simulink model "PLL1"  (R2021b)
settings: Solver=ode45  StartTime=0.0  StopTime=500*synM/synFr  FixedStep=1/(3*synFr*synN/synM)  MaxStep=.5/(synFr*synN/synM)  RelTol=1e-3  EnableMultiTasking=on
PreLoadFcn:
  | synM = 3;    % frequency division ratio
  | synN = 10;   % frequency division ratio
  | synFr = 30e6;   % reference frequency
  | synFq = synFr;       % quiescent frequency
  | synSen = 40e6;   % VCO sensitivity
libraries: commblksprivate x3, dsparch4 x1, commsynccomp2 x1
Description:
  | Phase-Locked Loop (PLL)  Based Frequency Synthesis
  | 
  | This model shows how to simulate a phase-locked loop (PLL) frequency synthesizer.
settings Model: Creator=The MathWorks, Inc.  LastModifiedBy=think
settings SolverCC: AlgebraicLoopSolver=TrustRegion
settings DataIOCC: LimitDataPoints=on  SaveFormat=Array  SaveOutput=off  SaveTime=off  ReturnWorkspaceOutputs=off  SignalLoggingName=synSigsOut
settings OptimizationCC: BlockReduction=off  BooleanDataType=off  ExpressionDepthLimit=2147483647  InitFltsAndDblsToZero=on  EfficientMapNaN2IntZero=off  LifeSpan=inf
settings DebuggingCC: SaveWithParameterizedLinksMsg=none  UnderspecifiedInitializationDetection=Classic  MergeDetectMultiDrivingBlocksExec=none  CheckExecutionContextPreStartOutputMsg=on  SignalResolutionControl=TryResolveAllWithWarning  MultiTaskDSMMsg=warning  MultiTaskCondExecSysMsg=none  SigSpecEnsureSampleTimeMsg=none  FcnCallInpInsideContextMsg=warning  AllowSymbolicDim=off  StateNameClashWarn=warning  SFUnexpectedBacktrackingDiag=warning  SFNoUnconditionalDefaultTransitionDiag=warning  SFMachineParentedDataDiag=warning  ArithmeticOperatorsInVariantConditions=warning
settings HardwareCC: ProdBitPerPointer=32  ProdBitPerSizeT=32  ProdBitPerPtrDiffT=32  ProdLargestAtomicFloat=None  ProdIntDivRoundTo=Undefined  ProdEndianess=Unspecified  ProdWordSize=32  ProdHWDeviceType=32-bit Generic  TargetUnknown=on
settings ModelReferenceCC: UpdateModelReferenceTargets=IfOutOfDate  PropagateSignalLabelsOutOfModel=off
settings SFSimCC: SimUseLocalCustomCode=off  CustomCodeUndefinedFunction=UseInterfaceOnly
settings RTWCC: RTWUseLocalCustomCode=off
settings CodeAppCC: StateflowObjectComments=on
settings GRTTargetCC: TargetFcnLib=ansi_tfl_tmw.mat  TargetLangStandard=C89/C90 (ANSI)  CombineOutputUpdateFcns=off  GRTInterface=on
settings ConfigComp: CovMetricSettings=d  CovSaveCumulativeToWorkspaceVar=on  CovSaveSingleToWorkspaceVar=on  CovExternalEMLEnable=off  CovSFcnEnable=off

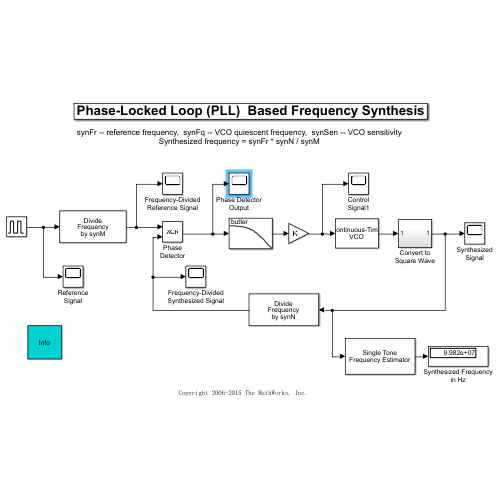
[thumbnail: Simulink's stored preview of the top-level diagram]
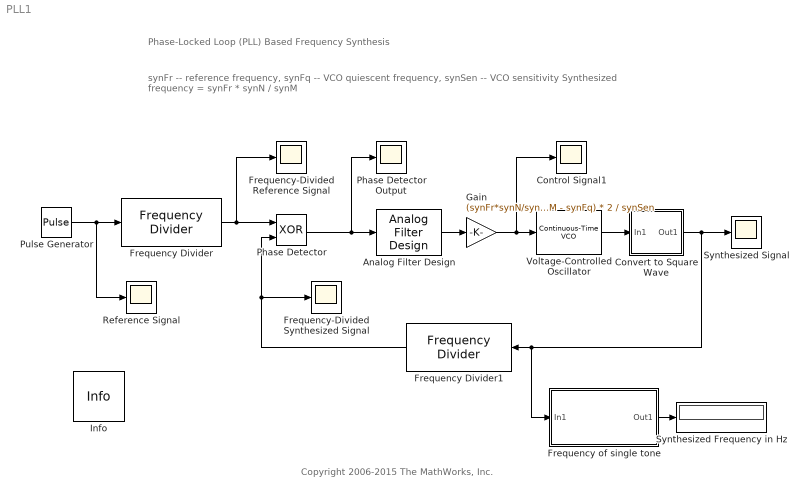
== system PLL1 ==
  note: Phase-Locked Loop (PLL) Based Frequency Synthesis
  note: synFr -- reference frequency,  synFq -- VCO quiescent frequency,  synSen -- VCO sensitivity
      | Synthesized frequency = synFr * synN / synM
  note: Copyright 2006-2015 The MathWorks, Inc.
  Analog Filter Design : dsparch4/Analog Filter Design  method=Butterworth  filttype=Lowpass  N=1  Wlo=synFr/synM/10  Whi=80  Rp=2  Rs=40
  Control Signal1 : Scope
  Convert to Square Wave : Subsystem
  Frequency Divider : commblksprivate/Frequency Divider  n=synM
      settings: SourceProductBaseCode=CM
  Frequency Divider1 : commblksprivate/Frequency Divider  n=synN
      settings: SourceProductBaseCode=CM
  Frequency of single tone : Subsystem
      mask Display: disp('Single Tone\nFrequency Estimator');
  Frequency-Divided Reference Signal : Scope
  Frequency-Divided Synthesized Signal : Scope
  Gain : Gain  Gain=(synFr*synN/synM - synFq) * 2 / synSen  SaturateOnIntegerOverflow=on  OutDataTypeStr=Inherit: Same as input  ParamDataTypeStr=Inherit: Same as input
  Info : commblksprivate/Info  SystemSampleTime=-1  VariantActivationTime=update diagram  Latency=0  AutoFrameSizeCalculation=off
      settings: SourceProductBaseCode=CM
  Phase Detector : Logic  Operator=XOR
  Phase Detector Output : Scope
  Pulse Generator : DiscretePulseGenerator  PulseType=Time based  Period=1/synFr  PulseWidth=50
  Reference Signal : Scope
  Synthesized Signal : Scope
  Synthesized Frequency in Hz : Display
  Voltage-Controlled Oscillator : commsynccomp2/Continuous-Time VCO  Ac=1  Fc=synFq  Kc=synSen  Ph=0
      settings: SourceProductBaseCode=CM
  wires:
  Pulse Generator/1 -> Reference Signal/1, Frequency Divider/1
  Phase Detector/1 -> Analog Filter Design/1, Phase Detector Output/1
  Gain/1 -> Control Signal1/1, Voltage-Controlled Oscillator/1
  Voltage-Controlled Oscillator/1 -> Convert to Square Wave/1(In1)
  Convert to Square Wave/1(Out1) -> Synthesized Signal/1, Frequency Divider1/1, Frequency of single tone/1(In1)
  Frequency Divider/1 -> Phase Detector/1, Frequency-Divided Reference Signal/1
  Frequency Divider1/1 -> Phase Detector/2, Frequency-Divided Synthesized Signal/1
  Analog Filter Design/1 -> Gain/1
  Frequency of single tone/1(Out1) -> Synthesized Frequency in Hz/1

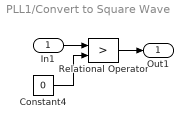
== system PLL1/Convert to Square Wave ==
  In1 : Inport
  Constant4 : Constant  Value=0
  Relational Operator : RelationalOperator  Operator=>  RndMeth=Nearest  InputSameDT=on
  Out1 : Outport
  wires:
  Relational Operator/1 -> Out1/1
  In1/1 -> Relational Operator/1
  Constant4/1 -> Relational Operator/2

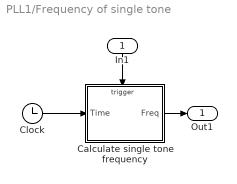
== system PLL1/Frequency of single tone ==
  In1 : Inport
  Calculate single tone frequency : Subsystem  TreatAsAtomicUnit=on
  Clock : Clock
  Out1 : Outport
  wires:
  Calculate single tone frequency/1(Freq) -> Out1/1
  Clock/1 -> Calculate single tone frequency/1(Time)
  In1/1 -> Calculate single tone frequency/Trigger

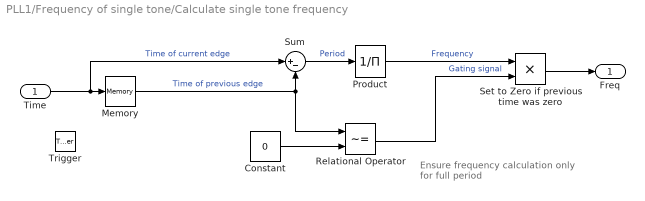
== system PLL1/Frequency of single tone/Calculate single tone frequency ==
  note: Ensure frequency calculation
      | only for full period
  Time : Inport
  Trigger : TriggerPort  VariantControl=Variant  ZeroCross=off
  Constant : Constant  Value=0
  Memory : Memory  InheritSampleTime=on
  Product : Product  Inputs=/  InputSameDT=on  SaturateOnIntegerOverflow=on  OutDataTypeStr=Inherit: Same as first input
  Relational Operator : RelationalOperator  Operator=~=  RndMeth=Nearest  InputSameDT=on
  Set to Zero if previous time was zero : Product  InputSameDT=on  SaturateOnIntegerOverflow=on  OutDataTypeStr=Inherit: Same as first input
  Sum : Sum  Inputs=|+-  InputSameDT=on  SaturateOnIntegerOverflow=on  OutDataTypeStr=Inherit: Same as first input
  Freq : Outport  InitialOutput=0
  wires:
  Relational Operator/1 -> Set to Zero if previous time was zero/2  "Gating signal"
  Constant/1 -> Relational Operator/2
  Set to Zero if previous time was zero/1 -> Freq/1
  Memory/1 -> Relational Operator/1, Sum/2  "Time of previous edge"
  Product/1 -> Set to Zero if previous time was zero/1  "Frequency"
  Sum/1 -> Product/1  "Period"
  Time/1 -> Memory/1, Sum/1  "Time of current edge"
